simulink model "4. To develop program modules based on operation on sequences like Signal addition, Signal multiplication, Signal fol"  (R2024b)
settings: Solver=VariableStepAuto  StartTime=0.0  StopTime=10  RelTol=1e-3  EnableMultiTasking=on
settings Model: Creator=CSE  LastModifiedBy=sobha
settings SolverCC: AlgebraicLoopSolver=TrustRegion
settings DataIOCC: ReturnWorkspaceOutputs=off
settings OptimizationCC: LifeSpan=inf
settings DebuggingCC: UnconnectedInputMsg=warning  UnconnectedOutputMsg=warning  UnconnectedLineMsg=warning  SFUnexpectedBacktrackingDiag=warning  SFNoUnconditionalDefaultTransitionDiag=warning  ArithmeticOperatorsInVariantConditions=warning
settings ModelReferenceCC: EnableRefExpFcnMdlSchedulingChecks=on
settings SFSimCC: SimUseLocalCustomCode=off  CustomCodeUndefinedFunction=UseInterfaceOnly
settings RTWCC: RTWUseLocalCustomCode=off  GPUComputeCapability=3.5
settings CodeAppCC: StateflowObjectComments=on
settings GRTTargetCC: TargetLangStandard=C89/C90 (ANSI)
settings ConfigComp: CovMetricSettings=dw  CovSaveCumulativeToWorkspaceVar=on  CovSaveSingleToWorkspaceVar=on  CovExternalEMLEnable=off

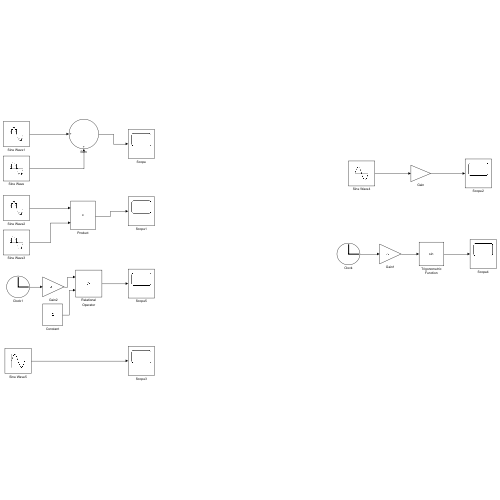
[thumbnail: Simulink's stored preview of the top-level diagram]
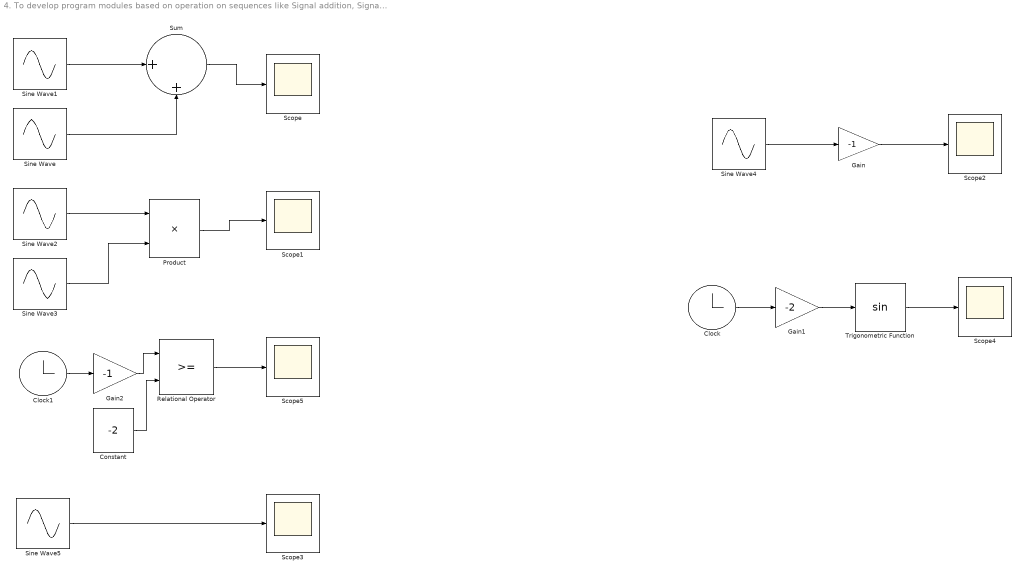
== system 4. To develop program modules based on operation on sequences like Signal addition, Signal multiplication, Signal fol ==
  Clock : Clock
  Clock1 : Clock
  Constant : Constant  Value=-2
  Gain : Gain  Gain=-1
  Gain1 : Gain  Gain=-2
  Gain2 : Gain  Gain=-1
  Product : Product
  Relational Operator : RelationalOperator  OutDataTypeStr=boolean  InputSameDT=off
  Scope{,1..5} (6 alike) : Scope
  Sine Wave : Sin  Frequency=2*pi*10  SampleTime=1e-4
  Sine Wave1 : Sin  Amplitude=2  Frequency=2*pi*5  SampleTime=1e-4
  Sine Wave2 : Sin  SampleTime=1e-4
  Sine Wave3 : Sin  Frequency=2*pi*10  SampleTime=1e-4
  Sine Wave4 : Sin  SampleTime=0
  Sine Wave5 : Sin  Phase=-1  SampleTime=0
  Sum : Sum  Inputs=|++
  Trigonometric Function : Trigonometry
  wires:
  Sine Wave1/1 -> Sum/1
  Sine Wave/1 -> Sum/2
  Sum/1 -> Scope/1
  Sine Wave2/1 -> Product/1
  Sine Wave3/1 -> Product/2
  Product/1 -> Scope1/1
  Sine Wave4/1 -> Gain/1
  Gain/1 -> Scope2/1
  Sine Wave5/1 -> Scope3/1
  Clock/1 -> Gain1/1
  Gain1/1 -> Trigonometric Function/1
  Trigonometric Function/1 -> Scope4/1
  Clock1/1 -> Gain2/1
  Gain2/1 -> Relational Operator/1
  Relational Operator/1 -> Scope5/1
  Constant/1 -> Relational Operator/2
